simulink model "AXU5EV_Encoder_Angle_HDL"  (R2026b)
settings: Solver=FixedStepDiscrete  StopTime=0.0001  FixedStep=2e-8
libraries: AXU5EV_Encoder_Components x1
settings Model: Creator=lww  LastModifiedBy=lww

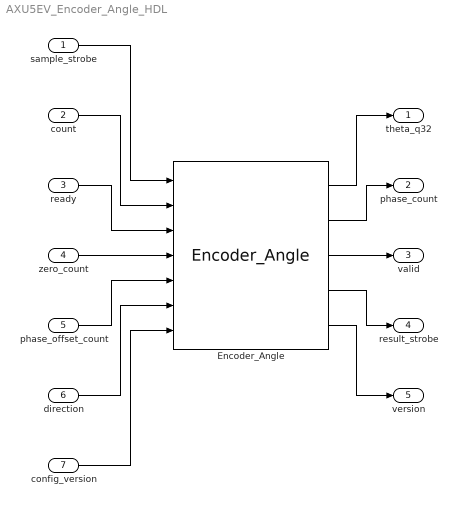
== system AXU5EV_Encoder_Angle_HDL ==
  sample_strobe : Inport  OutDataTypeStr=boolean  SampleTime=2e-8
  count : Inport  Port=2  OutDataTypeStr=uint32  SampleTime=2e-8
  ready : Inport  Port=3  OutDataTypeStr=boolean  SampleTime=2e-8
  zero_count : Inport  Port=4  OutDataTypeStr=uint32  SampleTime=2e-8
  phase_offset_count : Inport  Port=5  OutDataTypeStr=uint16  SampleTime=2e-8
  direction : Inport  Port=6  OutDataTypeStr=boolean  SampleTime=2e-8
  config_version : Inport  Port=7  OutDataTypeStr=uint32  SampleTime=2e-8
  Encoder_Angle : AXU5EV_Encoder_Components/Encoder_Angle  SystemSampleTime=-1  VariantActivationTime=update diagram  EmptyChoice=off  PassThrough=off  PassThroughVariantControl=(default)  EmptyChoiceVariantControl=(default)  AllowFlexibleInterface=on  Latency=0  AutoFrameSizeCalculation=off
  theta_q32 : Outport
  phase_count : Outport  Port=2
  valid : Outport  Port=3
  result_strobe : Outport  Port=4
  version : Outport  Port=5
  wires:
  Encoder_Angle/5 -> version/1
  Encoder_Angle/4 -> result_strobe/1
  Encoder_Angle/3 -> valid/1
  Encoder_Angle/2 -> phase_count/1
  Encoder_Angle/1 -> theta_q32/1
  config_version/1 -> Encoder_Angle/7
  direction/1 -> Encoder_Angle/6
  phase_offset_count/1 -> Encoder_Angle/5
  zero_count/1 -> Encoder_Angle/4
  ready/1 -> Encoder_Angle/3
  count/1 -> Encoder_Angle/2
  sample_strobe/1 -> Encoder_Angle/1
